simulink model "DTCSVM_compressor"  (R2024b)
settings: Solver=VariableStepAuto  StartTime=0.0  StopTime=1  RelTol=1e-3
values from neighbouring files (symbols this model uses):
  b = 1e-3    (= 0.001)    [BLDTCSVM_parameters.m]
  Cn = Pn / Wn    (= 17.0057056694)    [BLDTCSVM_parameters.m]
  Edc = 380    [BLDTCSVM_parameters.m]
  Fe = 0.1367    [BLDTCSVM_parameters.m]
  invD = D^(-1)    [BLDTCSVM_parameters.m]
  J = Jc+Jm    (= 0.0268)    [BLDTCSVM_parameters.m]
  Ki_f = 5000    [BLDTCSVM_parameters.m]
  Ki_s = 1    [BLDTCSVM_parameters.m]
  Ki_t = 10000    [BLDTCSVM_parameters.m]
  Kp_s = Ki_s*tau_m    (= 26.8)    [BLDTCSVM_parameters.m]
  Kp_t = Ki_t*tau_e    (= 141.35090683)    [BLDTCSVM_parameters.m]
  Ls = (Lmedio*1e-3)/2    (= 0.0063425)    [BLDTCSVM_parameters.m]
  Nn = 1200    [BLDTCSVM_parameters.m]
  p = 3    [BLDTCSVM_parameters.m]
  Rs = (0.628/2)*(1+(135-25)*3.9e-3)    (= 0.448706)    [BLDTCSVM_parameters.m]
  Tc = 50e-6    (= 5e-05)    [BLDTCSVM_parameters.m]
  theta_rad = deg2rad(theta_deg)    [BLDTCSVM_parameters.m]
  Torque = (Torque * 10) / max(Torque)    [BLDTCSVM_parameters.m]
undefined symbols (not defined in the file or in its folder): DiscIntNeverNeededParam
libraries: slpidlib x3
settings Model: Creator=Utente  LastModifiedBy=Utente

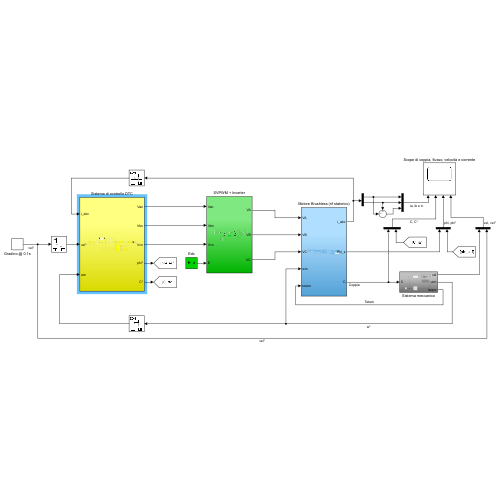
[thumbnail: Simulink's stored preview of the top-level diagram]
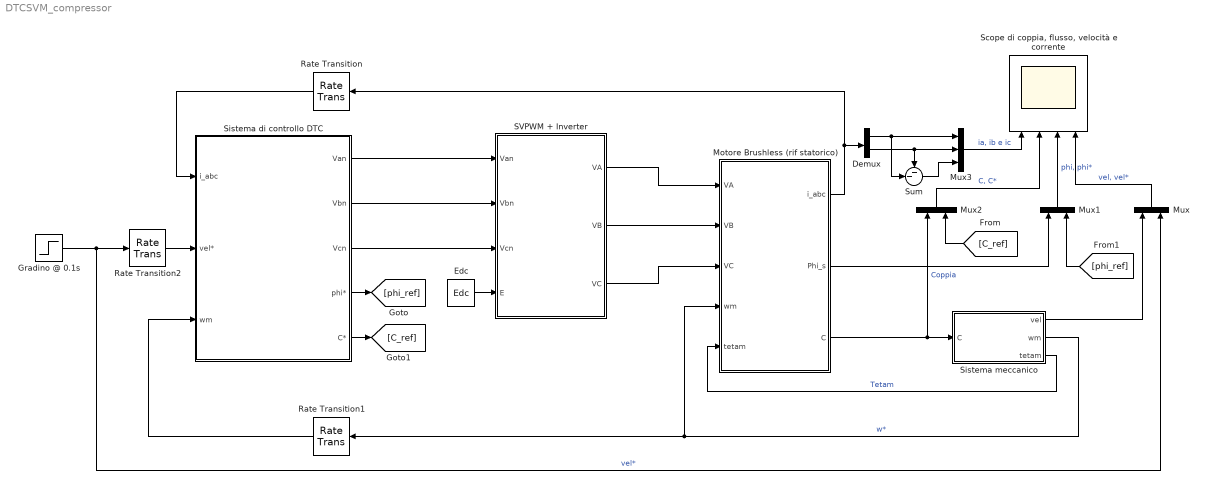
== system DTCSVM_compressor ==
  Demux : Demux  Outputs=2
  Edc : Constant  Value=Edc
  Gradino @ 0.1s : Step  Time=0.1  After=Nn  SampleTime=0
  Motore Brushless (rif statorico) : Subsystem
  Mux : Mux  Inputs=2
  Mux1 : Mux  Inputs=2
  Mux2 : Mux  Inputs=2
  Mux3 : Mux  Inputs=3
  Rate Transition : RateTransition  OutPortSampleTime=Tc
  Rate Transition1 : RateTransition  OutPortSampleTime=Tc
  Rate Transition2 : RateTransition  OutPortSampleTime=Tc
  SVPWM + Inverter : Subsystem
  "Scope di coppia, flusso, velocità e corrente" : Scope  NumInputPorts=4
  Sistema di controllo DTC : Subsystem
  Sistema meccanico : Subsystem
  Sum : Sum  Inputs=--|
  wires:
  Sistema meccanico/2(wm) -> Motore Brushless (rif statorico)/4(wm), Rate Transition1/1  "w*"
  SVPWM + Inverter/3(VC) -> Motore Brushless (rif statorico)/3(VC)
  Sistema meccanico/3(tetam) -> Motore Brushless (rif statorico)/5(tetam)  "Tetam"
  SVPWM + Inverter/1(VA) -> Motore Brushless (rif statorico)/1(VA)
  SVPWM + Inverter/2(VB) -> Motore Brushless (rif statorico)/2(VB)
  Edc/1 -> SVPWM + Inverter/4(E)
  Gradino @ 0.1s/1 -> Mux/2, Rate Transition2/1  "vel*"
  Sistema di controllo DTC/1(Van) -> SVPWM + Inverter/1(Van)
  Sistema di controllo DTC/2(Vbn) -> SVPWM + Inverter/2(Vbn)
  Sistema di controllo DTC/3(Vcn) -> SVPWM + Inverter/3(Vcn)
  Motore Brushless (rif statorico)/3(C) -> Mux2/1, Sistema meccanico/1(C)  "Coppia"
  Motore Brushless (rif statorico)/1(i_abc) -> Rate Transition/1, Demux/1
  Sistema meccanico/1(vel) -> Mux/1
  Demux/1 -> Sum/2, Mux3/1
  Demux/2 -> Sum/1, Mux3/2
  Sum/1 -> Mux3/3
  Motore Brushless (rif statorico)/2(Phi_s) -> Mux1/1
  Rate Transition/1 -> Sistema di controllo DTC/1(i_abc)
  Rate Transition1/1 -> Sistema di controllo DTC/3(wm)
  Rate Transition2/1 -> Sistema di controllo DTC/2(vel*)
  Sistema di controllo DTC/4(phi*) -> [phi_ref]
  Sistema di controllo DTC/5(C*) -> [C_ref]
  [C_ref] -> Mux2/2
  [phi_ref] -> Mux1/2
  Mux/1 -> "Scope di coppia, flusso, velocità e corrente"/4  "vel, vel*"
  Mux2/1 -> "Scope di coppia, flusso, velocità e corrente"/2  "C, C*"
  Mux1/1 -> "Scope di coppia, flusso, velocità e corrente"/3  "phi, phi*"
  Mux3/1 -> "Scope di coppia, flusso, velocità e corrente"/1  "ia, ib e ic"

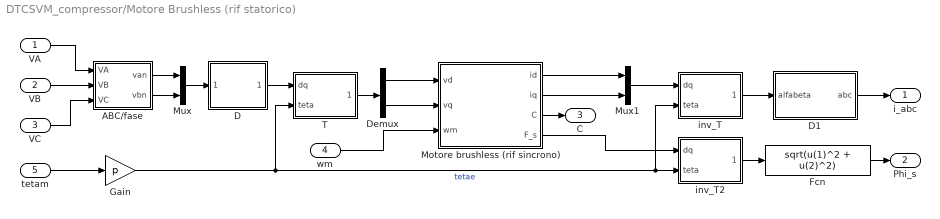
== system DTCSVM_compressor/Motore Brushless (rif statorico) ==
  VA : Inport
  VB : Inport  Port=2
  VC : Inport  Port=3
  wm : Inport  Port=4
  tetam : Inport  Port=5
  ABC/fase : Subsystem
  D : Subsystem
  D1 : Subsystem
  Demux : Demux  Outputs=2
  Fcn : Fcn  Expr=sqrt(u(1)^2 + u(2)^2)
  Gain : Gain  Gain=p
  Motore brushless (rif sincrono) : Subsystem
  Mux : Mux  Inputs=2
  Mux1 : Mux  Inputs=2
  T : Subsystem
  inv_T : Subsystem
  inv_T2 : Subsystem
  i_abc : Outport
  Phi_s : Outport  Port=2
  C : Outport  Port=3
  wires:
  Mux/1 -> D/1(ab(c))
  D/1(dq(0)) -> T/1(dq)
  tetam/1 -> Gain/1
  Gain/1 -> T/2(teta), inv_T2/2(teta), inv_T/2(teta)  "tetae"
  T/1(dq(teta)) -> Demux/1
  Demux/1 -> Motore brushless (rif sincrono)/1(vd)
  Demux/2 -> Motore brushless (rif sincrono)/2(vq)
  wm/1 -> Motore brushless (rif sincrono)/3(wm)
  Motore brushless (rif sincrono)/1(id) -> Mux1/1
  Motore brushless (rif sincrono)/2(iq) -> Mux1/2
  Mux1/1 -> inv_T/1(dq)
  Motore brushless (rif sincrono)/3(C) -> C/1
  VA/1 -> ABC/fase/1(VA)
  VB/1 -> ABC/fase/2(VB)
  VC/1 -> ABC/fase/3(VC)
  ABC/fase/1(van) -> Mux/1
  ABC/fase/2(vbn) -> Mux/2
  inv_T/1(alfa_beta) -> D1/1(alfabeta)
  Motore brushless (rif sincrono)/4(F_s) -> inv_T2/1(dq)
  inv_T2/1(alfa_beta) -> Fcn/1
  Fcn/1 -> Phi_s/1
  D1/1(abc) -> i_abc/1

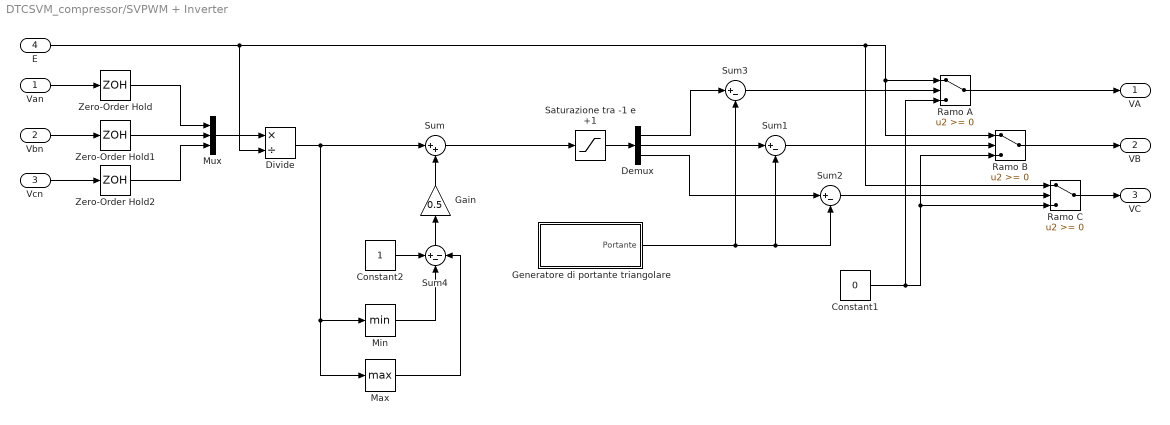
== system DTCSVM_compressor/SVPWM + Inverter ==
  Van : Inport
  Vbn : Inport  Port=2
  Vcn : Inport  Port=3
  E : Inport  Port=4
  Constant1 : Constant  Value=0
  Constant2 : Constant
  Demux : Demux  Outputs=3
  Divide : Product  Inputs=*/
  Gain : Gain  Gain=0.5
  Generatore di portante triangolare : Subsystem
  Max : MinMax  Function=max
  Min : MinMax
  Mux : Mux  Inputs=3
  Ramo A : Switch  SaturateOnIntegerOverflow=off  InputSameDT=off
  Ramo B : Switch  SaturateOnIntegerOverflow=off  InputSameDT=off
  Ramo C : Switch  SaturateOnIntegerOverflow=off  InputSameDT=off
  Saturazione tra -1 e +1 : Saturate  UpperLimit=1  LowerLimit=0
  Sum : Sum  Inputs=|++
  Sum1 : Sum  Inputs=|+-
  Sum2 : Sum  Inputs=|+-
  Sum3 : Sum  Inputs=|+-
  Sum4 : Sum  Inputs=+--
  Zero-Order Hold : ZeroOrderHold  SampleTime=Tc
  Zero-Order Hold1 : ZeroOrderHold  SampleTime=Tc
  Zero-Order Hold2 : ZeroOrderHold  SampleTime=Tc
  VA : Outport
  VB : Outport  Port=2
  VC : Outport  Port=3
  wires:
  Van/1 -> Zero-Order Hold/1
  Vbn/1 -> Zero-Order Hold1/1
  Vcn/1 -> Zero-Order Hold2/1
  Mux/1 -> Divide/1
  Saturazione tra -1 e +1/1 -> Demux/1
  Sum3/1 -> Ramo A/2
  Constant1/1 -> Ramo A/3, Ramo C/3, Ramo B/3
  Ramo A/1 -> VA/1
  Ramo C/1 -> VC/1
  Ramo B/1 -> VB/1
  Sum1/1 -> Ramo B/2
  Sum2/1 -> Ramo C/2
  Generatore di portante triangolare/1(Portante) -> Sum2/2, Sum1/2, Sum3/2
  Demux/1 -> Sum3/1
  Demux/2 -> Sum1/1
  Demux/3 -> Sum2/1
  E/1 -> Ramo A/1, Ramo B/1, Ramo C/1, Divide/2
  Zero-Order Hold/1 -> Mux/1
  Zero-Order Hold1/1 -> Mux/2
  Zero-Order Hold2/1 -> Mux/3
  Divide/1 -> Sum/1, Max/1, Min/1
  Min/1 -> Sum4/2
  Gain/1 -> Sum/2
  Sum4/1 -> Gain/1
  Sum/1 -> Saturazione tra -1 e +1/1
  Constant2/1 -> Sum4/1
  Max/1 -> Sum4/3

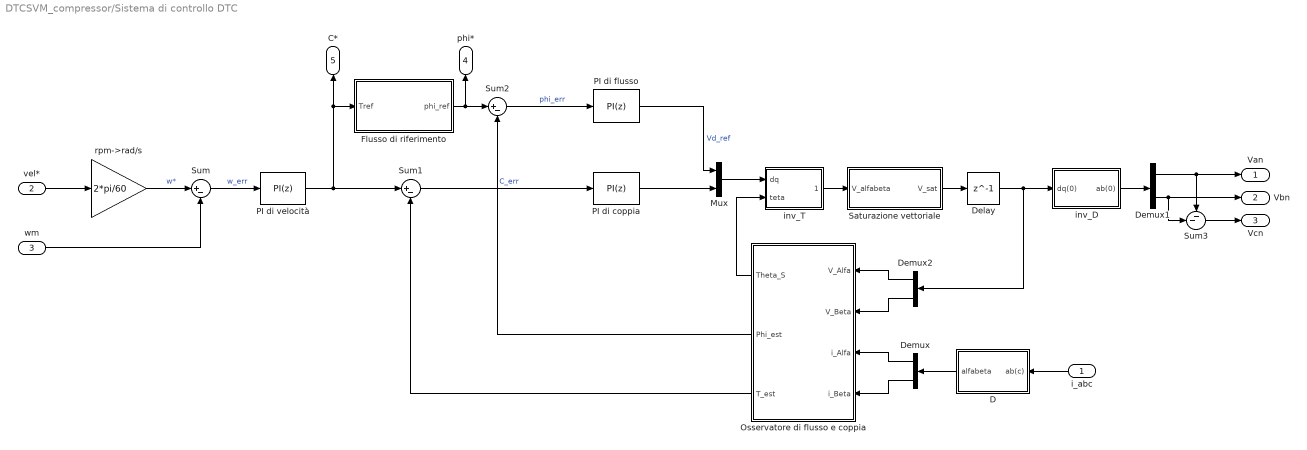
== system DTCSVM_compressor/Sistema di controllo DTC ==
  i_abc : Inport
  vel* : Inport  Port=2
  wm : Inport  Port=3
  D : Subsystem
  Delay : Delay  DelayLength=1  InitialCondition=0
  Demux : Demux  Outputs=2
  Demux1 : Demux  Outputs=2
  Demux2 : Demux  Outputs=2
  Flusso di riferimento : MATLAB Function  TreatAsAtomicUnit=on
  Mux : Mux  Inputs=2
  Osservatore di flusso e coppia : Subsystem
  PI di coppia : slpidlib/PID Controller  Controller=PI  Form=Parallel  TimeDomain=Discrete-time  UseExternalTs=off  SampleTime=Tc  IntegratorMethod=Forward Euler  FilterMethod=Forward Euler  ControllerParametersSource=internal  P=Kp_t  I=Ki_t  UseKiTs=off  D=0  UseExternalDerivativeSource=off  N=100  UseFilter=on  TunerSelectOption=Transfer Function Based (PID Tuner App)  InitialConditionSource=internal  InitialConditionForIntegrator=0  InitialConditionForFilter=0  DifferentiatorICPrevScaledInput=0  ExternalReset=none  TrackingMode=off  Kt=1  LimitOutput=off  SatLimitsSource=internal  UpperSaturationLimit=219  LowerSaturationLimit=-219  LinearizeAsGain=off  AntiWindupMode=clamping  Kb=1  LimitIntegrator=off  UpperIntegratorSaturationLimit=inf  LowerIntegratorSaturationLimit=-inf  POutMin=[]  POutMax=[]  IOutMin=[]  IOutMax=[]  DOutMin=[]  DOutMax=[]  NOutMin=[]  NOutMax=[]  SumOutMin=[]  SumOutMax=[]  SaturationOutMin=[]  SaturationOutMax=[]  PParamMin=[]  PParamMax=[]  IParamMin=[]  IParamMax=[]  DParamMin=[]  DParamMax=[]  NParamMin=[]  NParamMax=[]  KbParamMin=[]  KbParamMax=[]  KtParamMin=[]  KtParamMax=[]  KbOutMin=[]  KbOutMax=[]  KtOutMin=[]  KtOutMax=[]  IntegratorOutMin=[]  IntegratorOutMax=[]  FilterOutMin=[]  FilterOutMax=[]  SumI1OutMin=[]  SumI1OutMax=[]  SumI2OutMin=[]  SumI2OutMax=[]  SumI3OutMin=[]  SumI3OutMax=[]  SumI4OutMin=[]  SumI4OutMax=[]  SumDOutMin=[]  SumDOutMax=[]  DifferentiatorOutMin=[]  DifferentiatorOutMax=[]  FilterDiffOutCoefMin=[]  FilterDiffOutCoefMax=[]  ReciprocalOutMin=[]  ReciprocalOutMax=[]  SumDenOutMin=[]  SumDenOutMax=[]  SumNumOutMin=[]  SumNumOutMax=[]  DivideOutMin=[]  DivideOutMax=[]  UdiffTsProdOutMin=[]  UdiffTsProdOutMax=[]  NTsProdOutMin=[]  NTsProdOutMax=[]  UintegralTsProdOutMin=[]  UintegralTsProdOutMax=[]  UngainTsProdOutMin=[]  UngainTsProdOutMax=[]  ClampingZeroOutDataTypeStr=Inherit: Inherit via back propagation  ClampingZeroOutMin=[]  ClampingZeroOutMax=[]  FilterDenConstantOutDataTypeStr=Inherit: Inherit via back propagation  FilterDenConstantOutMin=[]  FilterDenConstantOutMax=[]  PCopyOutDataTypeStr=Inherit: Inherit via back propagation  PCopyOutMin=[]  PCopyOutMax=[]  NCopyOutDataTypeStr=Inherit: Inherit via back propagation  NCopyOutMin=[]  NCopyOutMax=[]  IntegratorContinuousStateAttributes=''  IntegratorStateMustResolveToSignalObject=off  IntegratorRTWStateStorageClass=Auto  FilterContinuousStateAttributes=''  FilterStateMustResolveToSignalObject=off  FilterRTWStateStorageClass=Auto  ParallelPVariant=InternalParameters  IdealPVariant=Disabled  IVariant=InternalParameters  DVariant=Disabled  IntegratorVariant=Discrete  SatVariant=Disabled  AWVariant=Passthrough  PCopyVariant=Disabled  TRVariant=Disabled  FdbkBlocksVariant=Forward  IdealPFdbkVariant=Disabled  SatFdbkVariant=Disabled  DerivativeFilterVariant=Disabled  NVariant=Disabled  NCopyVariant=Disabled_SignalSpec  FilterICVariant=Disabled  IntegratorICVariant=InternalICs  ExternalResetVariant=Disabled  TRSumVariant=Passthrough  SumFdbkVariant=Disabled  SumVariant=Sum_PI  TsampFilterVariant=InternalTs  TsampNgainVariant=Passthrough  TsampIntegralVariant=Disabled_SignalSpec  ExternalSaturationOutDataTypeStr=Inherit: Same as second input  DerivativeSourceVariant=Disabled  PreIntVariant=InternalPreInt
      settings: LibrarySourceBlock=simulink/Discrete/Discrete PID Controller
  PI di flusso : slpidlib/PID Controller  Controller=PI  Form=Parallel  TimeDomain=Discrete-time  UseExternalTs=off  SampleTime=Tc  IntegratorMethod=Forward Euler  FilterMethod=Forward Euler  ControllerParametersSource=internal  P=8000  I=Ki_f  UseKiTs=off  D=0  UseExternalDerivativeSource=off  N=100  UseFilter=on  TunerSelectOption=Transfer Function Based (PID Tuner App)  InitialConditionSource=internal  InitialConditionForIntegrator=Fe  InitialConditionForFilter=0  DifferentiatorICPrevScaledInput=0  ExternalReset=none  TrackingMode=off  Kt=1  LimitOutput=off  SatLimitsSource=internal  UpperSaturationLimit=219  LowerSaturationLimit=-219  LinearizeAsGain=off  AntiWindupMode=clamping  Kb=1  LimitIntegrator=off  UpperIntegratorSaturationLimit=inf  LowerIntegratorSaturationLimit=-inf  POutMin=[]  POutMax=[]  IOutMin=[]  IOutMax=[]  DOutMin=[]  DOutMax=[]  NOutMin=[]  NOutMax=[]  SumOutMin=[]  SumOutMax=[]  SaturationOutMin=[]  SaturationOutMax=[]  PParamMin=[]  PParamMax=[]  IParamMin=[]  IParamMax=[]  DParamMin=[]  DParamMax=[]  NParamMin=[]  NParamMax=[]  KbParamMin=[]  KbParamMax=[]  KtParamMin=[]  KtParamMax=[]  KbOutMin=[]  KbOutMax=[]  KtOutMin=[]  KtOutMax=[]  IntegratorOutMin=[]  IntegratorOutMax=[]  FilterOutMin=[]  FilterOutMax=[]  SumI1OutMin=[]  SumI1OutMax=[]  SumI2OutMin=[]  SumI2OutMax=[]  SumI3OutMin=[]  SumI3OutMax=[]  SumI4OutMin=[]  SumI4OutMax=[]  SumDOutMin=[]  SumDOutMax=[]  DifferentiatorOutMin=[]  DifferentiatorOutMax=[]  FilterDiffOutCoefMin=[]  FilterDiffOutCoefMax=[]  ReciprocalOutMin=[]  ReciprocalOutMax=[]  SumDenOutMin=[]  SumDenOutMax=[]  SumNumOutMin=[]  SumNumOutMax=[]  DivideOutMin=[]  DivideOutMax=[]  UdiffTsProdOutMin=[]  UdiffTsProdOutMax=[]  NTsProdOutMin=[]  NTsProdOutMax=[]  UintegralTsProdOutMin=[]  UintegralTsProdOutMax=[]  UngainTsProdOutMin=[]  UngainTsProdOutMax=[]  ClampingZeroOutDataTypeStr=Inherit: Inherit via back propagation  ClampingZeroOutMin=[]  ClampingZeroOutMax=[]  FilterDenConstantOutDataTypeStr=Inherit: Inherit via back propagation  FilterDenConstantOutMin=[]  FilterDenConstantOutMax=[]  PCopyOutDataTypeStr=Inherit: Inherit via back propagation  PCopyOutMin=[]  PCopyOutMax=[]  NCopyOutDataTypeStr=Inherit: Inherit via back propagation  NCopyOutMin=[]  NCopyOutMax=[]  IntegratorContinuousStateAttributes=''  IntegratorStateMustResolveToSignalObject=off  IntegratorRTWStateStorageClass=Auto  FilterContinuousStateAttributes=''  FilterStateMustResolveToSignalObject=off  FilterRTWStateStorageClass=Auto  ParallelPVariant=InternalParameters  IdealPVariant=Disabled  IVariant=InternalParameters  DVariant=Disabled  IntegratorVariant=Discrete  SatVariant=Disabled  AWVariant=Passthrough  PCopyVariant=Disabled  TRVariant=Disabled  FdbkBlocksVariant=Forward  IdealPFdbkVariant=Disabled  SatFdbkVariant=Disabled  DerivativeFilterVariant=Disabled  NVariant=Disabled  NCopyVariant=Disabled_SignalSpec  FilterICVariant=Disabled  IntegratorICVariant=InternalICs  ExternalResetVariant=Disabled  TRSumVariant=Passthrough  SumFdbkVariant=Disabled  SumVariant=Sum_PI  TsampFilterVariant=InternalTs  TsampNgainVariant=Passthrough  TsampIntegralVariant=Disabled_SignalSpec  ExternalSaturationOutDataTypeStr=Inherit: Same as second input  DerivativeSourceVariant=Disabled  PreIntVariant=InternalPreInt
      settings: LibrarySourceBlock=simulink/Discrete/Discrete PID Controller
  PI di velocità : slpidlib/PID Controller  Controller=PI  Form=Parallel  TimeDomain=Discrete-time  UseExternalTs=off  SampleTime=Tc  IntegratorMethod=Forward Euler  FilterMethod=Forward Euler  ControllerParametersSource=internal  P=Kp_s  I=Ki_s  UseKiTs=off  D=0.8  UseExternalDerivativeSource=off  N=2  UseFilter=off  TunerSelectOption=Transfer Function Based (PID Tuner App)  InitialConditionSource=internal  InitialConditionForIntegrator=0  InitialConditionForFilter=0  DifferentiatorICPrevScaledInput=0  ExternalReset=none  TrackingMode=off  Kt=1  LimitOutput=on  SatLimitsSource=internal  UpperSaturationLimit=Cn  LowerSaturationLimit=-Cn  LinearizeAsGain=off  AntiWindupMode=clamping  Kb=50  LimitIntegrator=off  UpperIntegratorSaturationLimit=inf  LowerIntegratorSaturationLimit=-inf  POutMin=[]  POutMax=[]  IOutMin=[]  IOutMax=[]  DOutMin=[]  DOutMax=[]  NOutMin=[]  NOutMax=[]  SumOutMin=[]  SumOutMax=[]  SaturationOutMin=[]  SaturationOutMax=[]  PParamMin=[]  PParamMax=[]  IParamMin=[]  IParamMax=[]  DParamMin=[]  DParamMax=[]  NParamMin=[]  NParamMax=[]  KbParamMin=[]  KbParamMax=[]  KtParamMin=[]  KtParamMax=[]  KbOutMin=[]  KbOutMax=[]  KtOutMin=[]  KtOutMax=[]  IntegratorOutMin=[]  IntegratorOutMax=[]  FilterOutMin=[]  FilterOutMax=[]  SumI1OutMin=[]  SumI1OutMax=[]  SumI2OutMin=[]  SumI2OutMax=[]  SumI3OutMin=[]  SumI3OutMax=[]  SumI4OutMin=[]  SumI4OutMax=[]  SumDOutMin=[]  SumDOutMax=[]  DifferentiatorOutMin=[]  DifferentiatorOutMax=[]  FilterDiffOutCoefMin=[]  FilterDiffOutCoefMax=[]  ReciprocalOutMin=[]  ReciprocalOutMax=[]  SumDenOutMin=[]  SumDenOutMax=[]  SumNumOutMin=[]  SumNumOutMax=[]  DivideOutMin=[]  DivideOutMax=[]  UdiffTsProdOutMin=[]  UdiffTsProdOutMax=[]  NTsProdOutMin=[]  NTsProdOutMax=[]  UintegralTsProdOutMin=[]  UintegralTsProdOutMax=[]  UngainTsProdOutMin=[]  UngainTsProdOutMax=[]  ClampingZeroOutDataTypeStr=Inherit: Inherit via back propagation  ClampingZeroOutMin=[]  ClampingZeroOutMax=[]  FilterDenConstantOutDataTypeStr=Inherit: Inherit via back propagation  FilterDenConstantOutMin=[]  FilterDenConstantOutMax=[]  PCopyOutDataTypeStr=Inherit: Inherit via back propagation  PCopyOutMin=[]  PCopyOutMax=[]  NCopyOutDataTypeStr=Inherit: Inherit via back propagation  NCopyOutMin=[]  NCopyOutMax=[]  IntegratorContinuousStateAttributes=''  IntegratorStateMustResolveToSignalObject=off  IntegratorRTWStateStorageClass=Auto  FilterContinuousStateAttributes=''  FilterStateMustResolveToSignalObject=off  FilterRTWStateStorageClass=Auto  ParallelPVariant=InternalParameters  IdealPVariant=Disabled  IVariant=InternalParameters  DVariant=Disabled  IntegratorVariant=Discrete  SatVariant=Enabled  AWVariant=DiscClampingParallel  PCopyVariant=Disabled  TRVariant=Disabled  FdbkBlocksVariant=Forward  IdealPFdbkVariant=Disabled  SatFdbkVariant=Disabled  DerivativeFilterVariant=Disabled  NVariant=Disabled  NCopyVariant=Disabled_SignalSpec  FilterICVariant=Disabled  IntegratorICVariant=InternalICs  ExternalResetVariant=Disabled  TRSumVariant=Passthrough  SumFdbkVariant=Disabled  SumVariant=Sum_PI  TsampFilterVariant=InternalTs  TsampNgainVariant=Passthrough  TsampIntegralVariant=Disabled_SignalSpec  ExternalSaturationOutDataTypeStr=Inherit: Same as second input  DerivativeSourceVariant=Disabled  PreIntVariant=InternalPreInt
      settings: LibrarySourceBlock=simulink/Discrete/Discrete PID Controller
  Saturazione vettoriale : Subsystem
  Sum : Sum  Inputs=|+-
  Sum1 : Sum  Inputs=|+-
  Sum2 : Sum  Inputs=|+-
  Sum3 : Sum  Inputs=--|
  inv_D : Subsystem
  inv_T : Subsystem
  rpm->rad/s : Gain  Gain=2*pi/60  SaturateOnIntegerOverflow=on  OutDataTypeStr=Inherit: Same as input  ParamDataTypeStr=Inherit: Same as input
  Van : Outport
  Vbn : Outport  Port=2
  Vcn : Outport  Port=3
  phi* : Outport  Port=4
  C* : Outport  Port=5
  wires:
  Sum1/1 -> PI di coppia/1  "C_err"
  Sum2/1 -> PI di flusso/1  "phi_err"
  inv_D/1(ab(0)) -> Demux1/1
  inv_T/1(dq(teta)) -> Saturazione vettoriale/1(V_alfabeta)
  Demux1/1 -> Sum3/1, Van/1
  Demux1/2 -> Sum3/2, Vbn/1
  Sum3/1 -> Vcn/1
  Mux/1 -> inv_T/1(dq)
  Flusso di riferimento/1(phi_ref) -> Sum2/1, phi*/1
  vel*/1 -> rpm->rad/s/1
  wm/1 -> Sum/2
  Demux2/1 -> Osservatore di flusso e coppia/1(V_Alfa)
  i_abc/1 -> D/1(ab(c))
  D/1(alfabeta) -> Demux/1
  Demux/1 -> Osservatore di flusso e coppia/3(i_Alfa)
  Demux/2 -> Osservatore di flusso e coppia/4(i_Beta)
  Saturazione vettoriale/1(V_sat) -> Delay/1
  Delay/1 -> Demux2/1, inv_D/1(dq(0))
  Demux2/2 -> Osservatore di flusso e coppia/2(V_Beta)
  Osservatore di flusso e coppia/1(Theta_S) -> inv_T/2(teta)
  Osservatore di flusso e coppia/2(Phi_est) -> Sum2/2
  Osservatore di flusso e coppia/3(T_est) -> Sum1/2
  rpm->rad/s/1 -> Sum/1  "w*"
  Sum/1 -> PI di velocità/1  "w_err"
  PI di velocità/1 -> C*/1, Flusso di riferimento/1(Tref), Sum1/1
  PI di coppia/1 -> Mux/2
  PI di flusso/1 -> Mux/1  "Vd_ref"

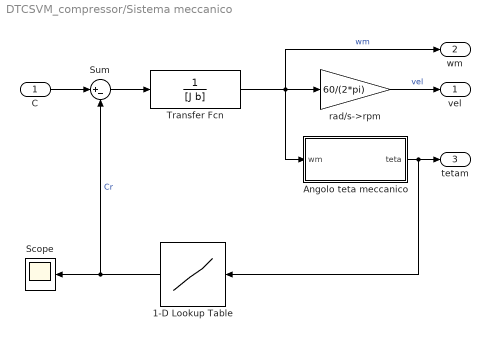
== system DTCSVM_compressor/Sistema meccanico ==
  C : Inport
  1-D Lookup Table : Lookup_n-D  NumberOfTableDimensions=1  BreakpointsForDimension1=theta_rad  Table=Torque  InternalRulePriority=Speed  RndMeth=Simplest
  Angolo teta meccanico : Subsystem
  Scope : Scope
  Sum : Sum  Inputs=|+-  InputSameDT=on  SaturateOnIntegerOverflow=on  OutDataTypeStr=Inherit: Same as first input
  Transfer Fcn : TransferFcn  Denominator=[J b]
  rad/s->rpm : Gain  Gain=60/(2*pi)  SaturateOnIntegerOverflow=on  OutDataTypeStr=Inherit: Same as input  ParamDataTypeStr=Inherit: Same as input
  vel : Outport
  wm : Outport  Port=2
  tetam : Outport  Port=3
  wires:
  C/1 -> Sum/1
  Sum/1 -> Transfer Fcn/1
  Transfer Fcn/1 -> wm/1, rad/s->rpm/1, Angolo teta meccanico/1(wm)  "wm"
  Angolo teta meccanico/1(teta) -> 1-D Lookup Table/1, tetam/1
  1-D Lookup Table/1 -> Scope/1, Sum/2  "Cr"
  rad/s->rpm/1 -> vel/1  "vel"

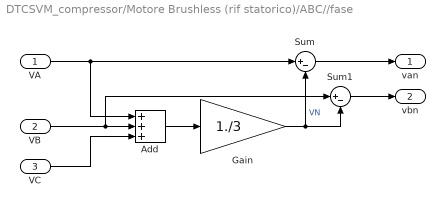
== system DTCSVM_compressor/Motore Brushless (rif statorico)/ABC//fase ==
  VA : Inport
  VB : Inport  Port=2
  VC : Inport  Port=3
  Add : Sum  Inputs=+++
  Gain : Gain  Gain=1./3
  Sum : Sum  Inputs=|+-
  Sum1 : Sum  Inputs=|+-
  van : Outport
  vbn : Outport  Port=2
  wires:
  VA/1 -> Add/1, Sum/1
  VB/1 -> Add/2, Sum1/1
  VC/1 -> Add/3
  Add/1 -> Gain/1
  Gain/1 -> Sum/2, Sum1/2  "VN"
  Sum/1 -> van/1
  Sum1/1 -> vbn/1

== system DTCSVM_compressor/Motore Brushless (rif statorico)/D ==
  ab(c) : Inport
  Gain : Gain  Gain=[1 0; 1/sqrt(3) 2/sqrt(3)]  Multiplication=Matrix(K*u)
  dq(0) : Outport
  wires:
  ab(c)/1 -> Gain/1
  Gain/1 -> dq(0)/1

== system DTCSVM_compressor/Motore Brushless (rif statorico)/D1 ==
  alfabeta : Inport
  Gain : Gain  Gain=invD  Multiplication=Matrix(K*u)
  abc : Outport
  wires:
  alfabeta/1 -> Gain/1
  Gain/1 -> abc/1

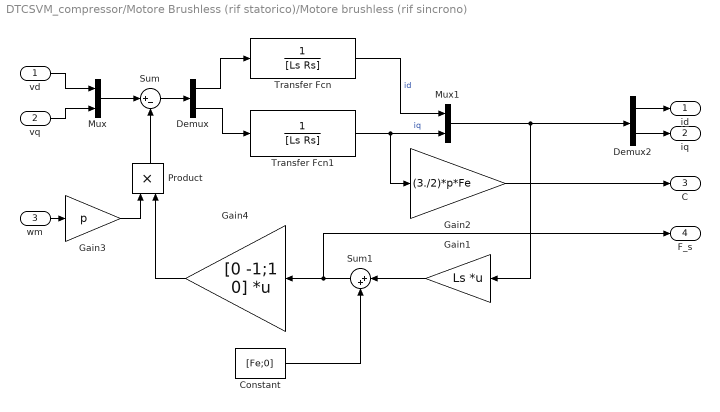
== system DTCSVM_compressor/Motore Brushless (rif statorico)/Motore brushless (rif sincrono) ==
  vd : Inport
  vq : Inport  Port=2
  wm : Inport  Port=3
  Constant : Constant  Value=[Fe;0]
  Demux : Demux  Outputs=2
  Demux2 : Demux  Outputs=2
  Gain1 : Gain  Gain=Ls  Multiplication=Matrix(K*u)  SaturateOnIntegerOverflow=on  OutDataTypeStr=Inherit: Same as input  ParamDataTypeStr=Inherit: Same as input
  Gain2 : Gain  Gain=(3./2)*p*Fe  SaturateOnIntegerOverflow=on  OutDataTypeStr=Inherit: Same as input  ParamDataTypeStr=Inherit: Same as input
  Gain3 : Gain  Gain=p  SaturateOnIntegerOverflow=on  OutDataTypeStr=Inherit: Same as input  ParamDataTypeStr=Inherit: Same as input
  Gain4 : Gain  Gain=[0 -1;1 0]  Multiplication=Matrix(K*u)  SaturateOnIntegerOverflow=on  OutDataTypeStr=Inherit: Same as input  ParamDataTypeStr=Inherit: Same as input
  Mux : Mux  Inputs=2
  Mux1 : Mux  Inputs=2
  Product : Product  RndMeth=Zero
  Sum : Sum  Inputs=|+-  InputSameDT=on  SaturateOnIntegerOverflow=on  OutDataTypeStr=Inherit: Same as first input
  Sum1 : Sum  Inputs=|++  InputSameDT=on  SaturateOnIntegerOverflow=on  OutDataTypeStr=Inherit: Same as first input
  Transfer Fcn : TransferFcn  Denominator=[Ls Rs]
  Transfer Fcn1 : TransferFcn  Denominator=[Ls Rs]
  id : Outport
  iq : Outport  Port=2
  C : Outport  Port=3
  F_s : Outport  Port=4
  wires:
  vd/1 -> Mux/1
  vq/1 -> Mux/2
  Mux/1 -> Sum/1
  Sum/1 -> Demux/1
  Demux/1 -> Transfer Fcn/1
  Demux/2 -> Transfer Fcn1/1
  Transfer Fcn/1 -> Mux1/1  "id"
  Transfer Fcn1/1 -> Mux1/2, Gain2/1  "iq"
  Mux1/1 -> Demux2/1, Gain1/1
  Gain4/1 -> Product/2
  Product/1 -> Sum/2
  Demux2/1 -> id/1
  Demux2/2 -> iq/1
  Sum1/1 -> F_s/1, Gain4/1
  Gain1/1 -> Sum1/1
  Constant/1 -> Sum1/2
  Gain2/1 -> C/1
  wm/1 -> Gain3/1
  Gain3/1 -> Product/1

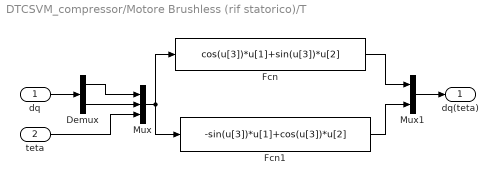
== system DTCSVM_compressor/Motore Brushless (rif statorico)/T ==
  dq : Inport
  teta : Inport  Port=2
  Demux : Demux  Outputs=2
  Fcn : Fcn  Expr=cos(u[3])*u[1]+sin(u[3])*u[2]
  Fcn1 : Fcn  Expr=-sin(u[3])*u[1]+cos(u[3])*u[2]
  Mux : Mux  Inputs=3
  Mux1 : Mux  Inputs=2
  dq(teta) : Outport
  wires:
  dq/1 -> Demux/1
  Demux/1 -> Mux/1
  Demux/2 -> Mux/2
  teta/1 -> Mux/3
  Mux/1 -> Fcn/1, Fcn1/1
  Fcn/1 -> Mux1/1
  Fcn1/1 -> Mux1/2
  Mux1/1 -> dq(teta)/1

== system DTCSVM_compressor/Motore Brushless (rif statorico)/inv_T ==
  dq : Inport
  teta : Inport  Port=2
  Gain : Gain  Gain=-1
  T : Subsystem
  alfa_beta : Outport
  wires:
  dq/1 -> T/1(dq)
  teta/1 -> Gain/1
  Gain/1 -> T/2(teta)
  T/1(dq(teta)) -> alfa_beta/1

== system DTCSVM_compressor/Motore Brushless (rif statorico)/inv_T2 ==
  dq : Inport
  teta : Inport  Port=2
  Gain : Gain  Gain=-1
  T : Subsystem
  alfa_beta : Outport
  wires:
  dq/1 -> T/1(dq)
  teta/1 -> Gain/1
  Gain/1 -> T/2(teta)
  T/1(dq(teta)) -> alfa_beta/1

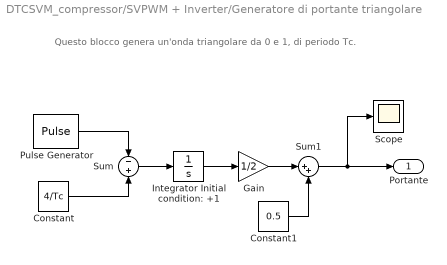
== system DTCSVM_compressor/SVPWM + Inverter/Generatore di portante triangolare ==
  note: Questo blocco genera un'onda triangolare da 0 e 1, di periodo Tc.
  Constant : Constant  Value=4/Tc
  Constant1 : Constant  Value=0.5
  Gain : Gain  Gain=1/2
  Integrator Initial condition: +1 : Integrator  InitialCondition=1
  Pulse Generator : DiscretePulseGenerator  PulseType=Time based  Amplitude=8/Tc  Period=Tc  PulseWidth=50
  Scope : Scope
  Sum : Sum  Inputs=-+
  Sum1 : Sum  Inputs=|++
  Portante : Outport
  wires:
  Sum/1 -> Integrator Initial condition: +1/1
  Pulse Generator/1 -> Sum/1
  Constant/1 -> Sum/2
  Integrator Initial condition: +1/1 -> Gain/1
  Gain/1 -> Sum1/1
  Sum1/1 -> Scope/1, Portante/1
  Constant1/1 -> Sum1/2

== system DTCSVM_compressor/Sistema di controllo DTC/D ==
  ab(c) : Inport
  Gain : Gain  Gain=[1 0; 1/sqrt(3) 2/sqrt(3)]  Multiplication=Matrix(K*u)
  alfabeta : Outport
  wires:
  ab(c)/1 -> Gain/1
  Gain/1 -> alfabeta/1

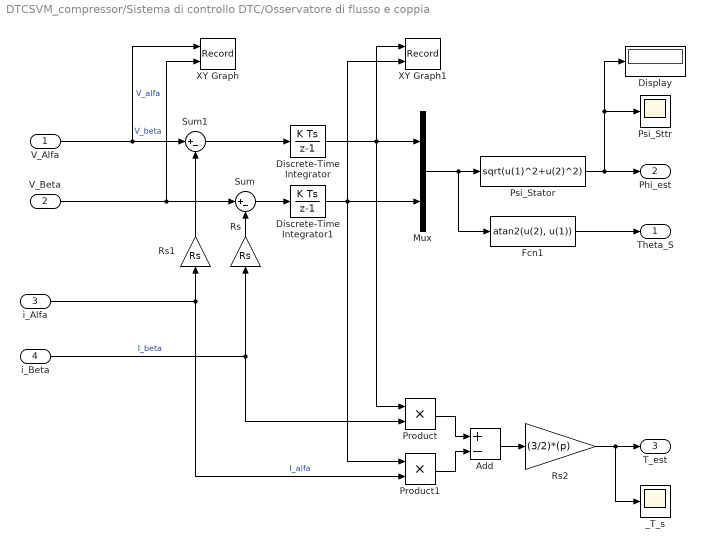
== system DTCSVM_compressor/Sistema di controllo DTC/Osservatore di flusso e coppia ==
  V_Alfa : Inport
  V_Beta : Inport  Port=2
  i_Alfa : Inport  Port=3
  i_Beta : Inport  Port=4
  Add : Sum  Inputs=+-
  Discrete-Time Integrator : DiscreteIntegrator  InitialCondition=Fe  SampleTime=Tc  ICPrevOutput=DiscIntNeverNeededParam  ICPrevScaledInput=DiscIntNeverNeededParam
  Discrete-Time Integrator1 : DiscreteIntegrator  SampleTime=Tc  ICPrevOutput=DiscIntNeverNeededParam  ICPrevScaledInput=DiscIntNeverNeededParam
  Display : Display
  Fcn1 : Fcn  Expr=atan2(u(2), u(1))
  Mux : Mux  Inputs=2
  Product : Product
  Product1 : Product
  Psi_Stator : Fcn  Expr=sqrt(u(1)^2+u(2)^2)
  Psi_Sttr : Scope
  Rs : Gain  Gain=Rs
  Rs1 : Gain  Gain=Rs
  Rs2 : Gain  Gain=(3/2)*(p)
  Sum : Sum  Inputs=|+-
  Sum1 : Sum  Inputs=|+-
  XY Graph : Record  FileSettingsInternal="{\"entries\":[{\"content\":{\"excelSettings\":{\"content\":{},\"type\":\"Streamout.ExcelSettings\"}},\"type\":\"Streamout.FileSettingStorage\",\"uuid\":\"\"}],\"packageUris\":[\"http:\\/\\/schema.mathworks.com\\/mf0\\/streamout_blocks\\/R2020a\"],\"version\":\"1.0\"}"  Layout=[1 1]  SignalsInternal="{\"entries\":[{\"content\":{\"signals\":[{\"content\":{\"blockPath\":[],\"dimensions\":[1],\"domain\":\"\",\"lineColor\":\"#a2142f\",\"plots\":[ 1 ],\"port\":1,\"sid\":[\"\"],\"signalID\":1,\"signalName\":\"V_alfa\"},\"type\":\"RecordBlkView.Signal\",\"uuid\":\"\"},{\"content\":{\"blockPath\":[],\"dimensions\":[1],\"domain\":\"\",\"lineColor\":\"#139fff\",\"plots\":[ 1 ],\"port\":2,\"sid\":[\"\"],\"signalID\":2,\"signalName\":\"V_beta\"},\"type\":\"RecordBlkView.Signal\",\"uuid\":\"\"}]},\"type\":\"RecordBlkView.InputSignals\",\"uuid\":\"\"}],\"packageUris\":[\"http:\\/\\/schema.mathworks.com\\/mf0\\/streamout_blocks\\/R2020a\"],\"version\":\"1.0\"}"  VisualizationBindings="{\"xyplotplugin\":{\"info\":[{\"series\":[{\"bindingParametersList\":[{\"parameter\":\"X-Axis\",\"signalID\":1,\"signalName\":\"V_alfa\"},{\"parameter\":\"Y-Axis\",\"signalID\":2,\"signalName\":\"V_beta\"}],\"seriesID\":0}],\"subplotID\":1}]}}"  CompatibilityTag=XY
  XY Graph1 : Record  FileSettingsInternal="{\"entries\":[{\"content\":{\"excelSettings\":{\"content\":{},\"type\":\"Streamout.ExcelSettings\"}},\"type\":\"Streamout.FileSettingStorage\",\"uuid\":\"\"}],\"packageUris\":[\"http:\\/\\/schema.mathworks.com\\/mf0\\/streamout_blocks\\/R2020a\"],\"version\":\"1.0\"}"  Layout=[1 1]  SignalsInternal="{\"entries\":[{\"content\":{\"signals\":[{\"content\":{\"blockPath\":[],\"dimensions\":[1],\"domain\":\"\",\"lineColor\":\"#a2142f\",\"plots\":[ 1 ],\"port\":1,\"sid\":[\"\"],\"signalID\":1,\"signalName\":\"Discrete-Time\\nIntegrator\"},\"type\":\"RecordBlkView.Signal\",\"uuid\":\"\"},{\"content\":{\"blockPath\":[],\"dimensions\":[1],\"domain\":\"\",\"lineColor\":\"#139fff\",\"plots\":[ 1 ],\"port\":2,\"sid\":[\"\"],\"signalID\":2,\"signalName\":\"Discrete-Time\\nIntegrator1\"},\"type\":\"RecordBlkView.Signal\",\"uuid\":\"\"}]},\"type\":\"RecordBlkView.InputSignals\",\"uuid\":\"\"}],\"packageUris\":[\"http:\\/\\/schema.mathworks.com\\/mf0\\/streamout_blocks\\/R2020a\"],\"version\":\"1.0\"}"  VisualizationBindings="{\"xyplotplugin\":{\"info\":[{\"series\":[{\"bindingParametersList\":[{\"parameter\":\"X-Axis\",\"signalID\":1,\"signalName\":\"Discrete-Time\\nIntegrator\"},{\"parameter\":\"Y-Axis\",\"signalID\":2,\"signalName\":\"Discrete-Time\\nIntegrator1\"}],\"seriesID\":0}],\"subplotID\":1}]}}"  CompatibilityTag=XY
  _T_s : Scope
  Theta_S : Outport
  Phi_est : Outport  Port=2
  T_est : Outport  Port=3
  wires:
  Rs/1 -> Sum/2
  Rs1/1 -> Sum1/2
  Sum1/1 -> Discrete-Time Integrator/1
  Mux/1 -> Fcn1/1, Psi_Stator/1
  Discrete-Time Integrator1/1 -> XY Graph1/2, Mux/2, Product1/1
  Product/1 -> Add/1
  Product1/1 -> Add/2
  Add/1 -> Rs2/1
  Psi_Stator/1 -> Display/1, Psi_Sttr/1, Phi_est/1
  Rs2/1 -> T_est/1, _T_s/1
  Discrete-Time Integrator/1 -> XY Graph1/1, Product/1, Mux/1
  V_Alfa/1 -> XY Graph/1, Sum1/1  "V_alfa"
  i_Alfa/1 -> Product1/2, Rs1/1  "I_alfa"
  Sum/1 -> Discrete-Time Integrator1/1
  i_Beta/1 -> Product/2, Rs/1  "I_beta"
  V_Beta/1 -> XY Graph/2, Sum/1  "V_beta"
  Fcn1/1 -> Theta_S/1

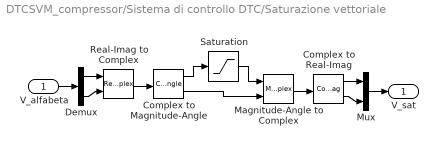
== system DTCSVM_compressor/Sistema di controllo DTC/Saturazione vettoriale ==
  V_alfabeta : Inport
  Complex to Magnitude-Angle : ComplexToMagnitudeAngle
  Complex to Real-Imag : ComplexToRealImag
  Demux : Demux  Outputs=2
  Magnitude-Angle to Complex : MagnitudeAngleToComplex
  Mux : Mux  Inputs=2
  Real-Imag to Complex : RealImagToComplex
  Saturation : Saturate  UpperLimit=Edc/sqrt(3)  LowerLimit=0
  V_sat : Outport
  wires:
  V_alfabeta/1 -> Demux/1
  Demux/1 -> Real-Imag to Complex/1
  Demux/2 -> Real-Imag to Complex/2
  Real-Imag to Complex/1 -> Complex to Magnitude-Angle/1
  Complex to Magnitude-Angle/2 -> Magnitude-Angle to Complex/2
  Magnitude-Angle to Complex/1 -> Complex to Real-Imag/1
  Complex to Real-Imag/1 -> Mux/1
  Complex to Real-Imag/2 -> Mux/2
  Mux/1 -> V_sat/1
  Complex to Magnitude-Angle/1 -> Saturation/1
  Saturation/1 -> Magnitude-Angle to Complex/1

== system DTCSVM_compressor/Sistema di controllo DTC/inv_D ==
  dq(0) : Inport
  Gain : Gain  Gain=invD  Multiplication=Matrix(K*u)
  ab(0) : Outport
  wires:
  dq(0)/1 -> Gain/1
  Gain/1 -> ab(0)/1

== system DTCSVM_compressor/Sistema di controllo DTC/inv_T ==
  dq : Inport
  teta : Inport  Port=2
  Gain1 : Gain  Gain=-1
  T : Subsystem
  dq(teta) : Outport
  wires:
  dq/1 -> T/1(dq)
  teta/1 -> Gain1/1
  T/1(dq(teta)) -> dq(teta)/1
  Gain1/1 -> T/2(teta)

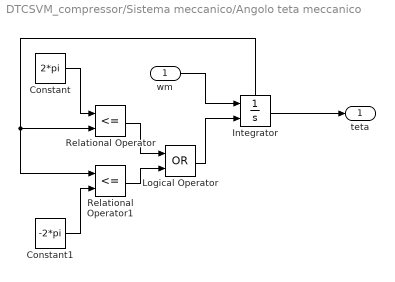
== system DTCSVM_compressor/Sistema meccanico/Angolo teta meccanico ==
  wm : Inport
  Constant : Constant  Value=2*pi
  Constant1 : Constant  Value=-2*pi
  Integrator : Integrator  ExternalReset=rising  ShowStatePort=on
  Logical Operator : Logic  Operator=OR  AllPortsSameDT=off  OutDataTypeStr=boolean
  Relational Operator : RelationalOperator  Operator=<=  OutDataTypeStr=boolean  InputSameDT=off
  Relational Operator1 : RelationalOperator  Operator=<=  OutDataTypeStr=boolean  InputSameDT=off
  teta : Outport
  wires:
  Integrator/1 -> teta/1
  Logical Operator/1 -> Integrator/2
  Relational Operator/1 -> Logical Operator/1
  Relational Operator1/1 -> Logical Operator/2
  wm/1 -> Integrator/1
  Integrator/State -> Relational Operator1/1, Relational Operator/2
  Constant/1 -> Relational Operator/1
  Constant1/1 -> Relational Operator1/2

== system DTCSVM_compressor/Motore Brushless (rif statorico)/inv_T/T ==
  dq : Inport
  teta : Inport  Port=2
  Demux : Demux  Outputs=2
  Fcn : Fcn  Expr=cos(u[3])*u[1]+sin(u[3])*u[2]
  Fcn1 : Fcn  Expr=-sin(u[3])*u[1]+cos(u[3])*u[2]
  Mux : Mux  Inputs=3
  Mux1 : Mux  Inputs=2
  dq(teta) : Outport
  wires:
  dq/1 -> Demux/1
  Demux/1 -> Mux/1
  Demux/2 -> Mux/2
  teta/1 -> Mux/3
  Mux/1 -> Fcn/1, Fcn1/1
  Fcn/1 -> Mux1/1
  Fcn1/1 -> Mux1/2
  Mux1/1 -> dq(teta)/1

== system DTCSVM_compressor/Motore Brushless (rif statorico)/inv_T2/T ==
  dq : Inport
  teta : Inport  Port=2
  Demux : Demux  Outputs=2
  Fcn : Fcn  Expr=cos(u[3])*u[1]+sin(u[3])*u[2]
  Fcn1 : Fcn  Expr=-sin(u[3])*u[1]+cos(u[3])*u[2]
  Mux : Mux  Inputs=3
  Mux1 : Mux  Inputs=2
  dq(teta) : Outport
  wires:
  dq/1 -> Demux/1
  Demux/1 -> Mux/1
  Demux/2 -> Mux/2
  teta/1 -> Mux/3
  Mux/1 -> Fcn/1, Fcn1/1
  Fcn/1 -> Mux1/1
  Fcn1/1 -> Mux1/2
  Mux1/1 -> dq(teta)/1

== system DTCSVM_compressor/Sistema di controllo DTC/inv_T/T ==
  dq : Inport
  teta : Inport  Port=2
  Demux : Demux  Outputs=2
  Fcn : Fcn  Expr=cos(u[3])*u[1]+sin(u[3])*u[2]
  Fcn1 : Fcn  Expr=-sin(u[3])*u[1]+cos(u[3])*u[2]
  Mux : Mux  Inputs=3
  Mux1 : Mux  Inputs=2
  dq(teta) : Outport
  wires:
  dq/1 -> Demux/1
  Demux/1 -> Mux/1
  Demux/2 -> Mux/2
  teta/1 -> Mux/3
  Mux/1 -> Fcn/1, Fcn1/1
  Fcn/1 -> Mux1/1
  Fcn1/1 -> Mux1/2
  Mux1/1 -> dq(teta)/1

== matlab function DTCSVM_compressor/Sistema di controllo DTC/Flusso di riferimento ==
  data: Tref input; phi_ref output; Fe parameter size=1; Ls parameter size=1; p parameter size=1
function phi_ref = MATLAB_Function(Tref, Fe, Ls, p)


phi_ref = sqrt(Fe^2 + ((Ls*2/(3*p*Fe))^2) * Tref^2 );
